simulink model "hybrid_system"  (R2026b)
settings: Solver=ode15s  StartTime=0  StopTime=200  MaxStep=0.01
undefined symbols (not defined in the file or in its folder): p
libraries: slpidlib x3
settings Model: Creator=ian  LastModifiedBy=hk

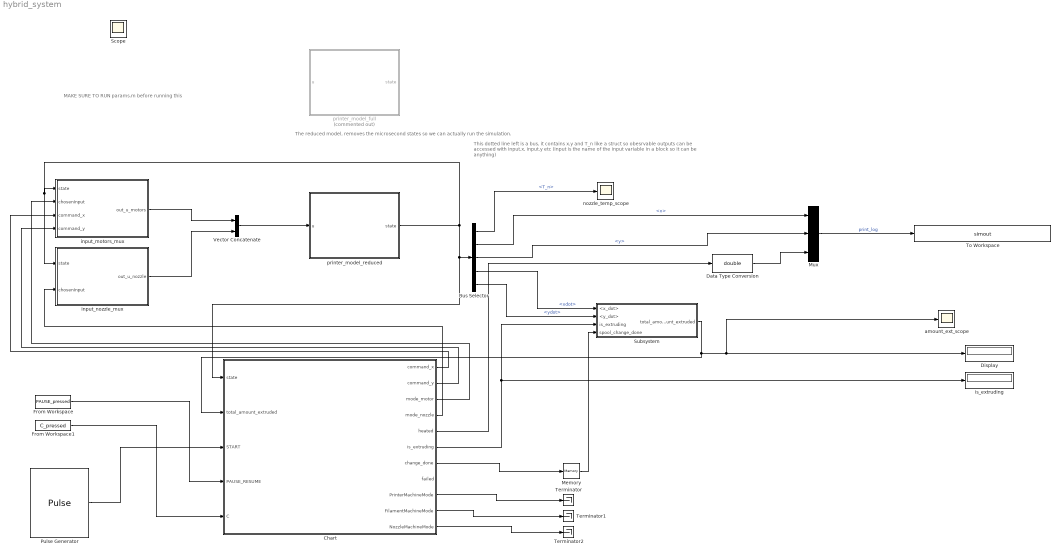
== system hybrid_system ==
  note: MAKE SURE TO RUN params.m before running this
  note: This dotted line left is a bus, it contains x,y and T_n like a struct so obesrvable outputs can be accessed with input.x, input.y etc (input is the name of the input variable in a block so it can be anything)
  note: The reduced model, removes the microsecond states so we can actually run the simulation.
  Bus Selector : BusSelector  OutputSignals=T_n,x,y,xdot,ydot
  Chart : Stateflow chart  TreatAsAtomicUnit=on
  Data Type Conversion : DataTypeConversion  OutDataTypeStr=double  SaturateOnIntegerOverflow=off  RndMeth=Floor
  Display : Display
  From Workspace : FromWorkspace  VariableName=PAUSE_pressed  Interpolate=off  OutputAfterFinalValue=Holding final value
  From Workspace1 : FromWorkspace  VariableName=C_pressed  Interpolate=off  OutputAfterFinalValue=Holding final value
  Memory : Memory
  Mux : Mux  Inputs=3
  Pulse Generator : DiscretePulseGenerator  PulseType=Time based  Period=1000  PulseWidth=0.5  PhaseDelay=1
  Subsystem : Subsystem
  Terminator : Terminator
  Terminator1 : Terminator
  Terminator2 : Terminator
  To Workspace : ToWorkspace  VariableName=simout  SaveFormat=Timeseries  SampleTime=-1
  Vector Concatenate : Concatenate
  amount_ext_scope : Scope
      settings: ActiveDisplayYMinimum=-54.541035477744657  ActiveDisplayYMaximum=83.193841611609969
  input_motors_mux : Subsystem
  input_nozzle_mux : Subsystem
  is_extruding : Display
  nozzle_temp_scope : Scope
      settings: ActiveDisplayYMinimum=258.016424423675  ActiveDisplayYMaximum=353.14399996630135
  printer_model_full : Subsystem  Commented=on
  printer_model_reduced : Subsystem
  Scope : Scope
      settings: DataLoggingVariableName=ScopeData2
  wires:
  Chart/4(mode_nozzle) -> input_nozzle_mux/2(chosenInput)
  printer_model_reduced/1(state) -> input_nozzle_mux/1(state), input_motors_mux/1(state), Chart/1(state), Bus Selector/1
  Bus Selector/1 -> nozzle_temp_scope/1  "<T_n>"
  Chart/3(mode_motor) -> input_motors_mux/2(chosenInput)
  input_nozzle_mux/1(out_u_nozzle) -> Vector Concatenate/2
  Vector Concatenate/1 -> printer_model_reduced/1(u)
  input_motors_mux/1(out_u_motors) -> Vector Concatenate/1
  Bus Selector/2 -> Mux/1  "<x>"
  Bus Selector/3 -> Mux/2  "<y>"
  Chart/5(heated) -> Data Type Conversion/1
  Data Type Conversion/1 -> Mux/3
  Mux/1 -> To Workspace/1  "print_log"
  Subsystem/1(total_amount_extruded) -> amount_ext_scope/1, Display/1, Chart/2(total_amount_extruded)
  Chart/1(command_x) -> input_motors_mux/3(command_x)
  Chart/2(command_y) -> input_motors_mux/4(command_y)
  Pulse Generator/1 -> Chart/3(START)
  From Workspace/1 -> Chart/4(PAUSE_RESUME)
  From Workspace1/1 -> Chart/5(C)
  Bus Selector/4 -> Subsystem/1(<x_dot>)  "<xdot>"
  Bus Selector/5 -> Subsystem/2(<y_dot>)  "<ydot>"
  Chart/7(change_done) -> Memory/1
  Memory/1 -> Subsystem/4(spool_change_done)
  Chart/6(is_extruding) -> is_extruding/1, Subsystem/3(is_extruding)
  Chart/9(" PrinterMachineMode") -> Terminator/1
  Chart/10(" FilamentMachineMode") -> Terminator1/1
  Chart/11(" NozzleMachineMode") -> Terminator2/1

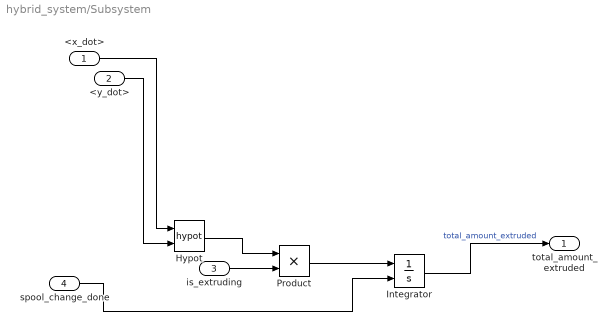
== system hybrid_system/Subsystem ==
  <x_dot> : Inport
  <y_dot> : Inport  Port=2
  is_extruding : Inport  Port=3
  spool_change_done : Inport  Port=4
  Hypot : Math  Operator=hypot
  Integrator : Integrator  ExternalReset=rising
  Product : Product
  total_amount_extruded : Outport
  wires:
  Hypot/1 -> Product/1
  Product/1 -> Integrator/1
  <y_dot>/1 -> Hypot/2
  is_extruding/1 -> Product/2
  <x_dot>/1 -> Hypot/1
  Integrator/1 -> total_amount_extruded/1  "total_amount_extruded"
  spool_change_done/1 -> Integrator/2

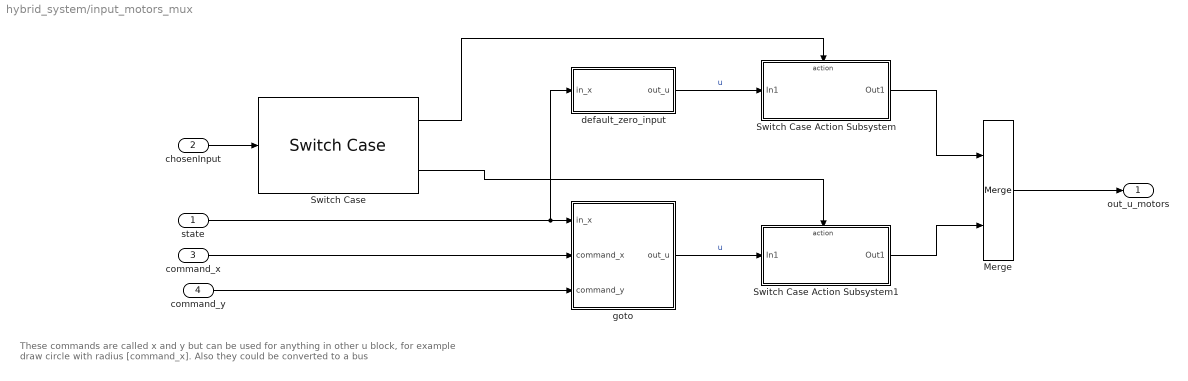
== system hybrid_system/input_motors_mux ==
  note: These commands are called x and y but can be used for anything in other u block, for example draw circle with radius [command_x]. Also they could be converted to a bus
  state : Inport
  chosenInput : Inport  Port=2  OutDataTypeStr=Enum: ModeMotors
  command_x : Inport  Port=3
  command_y : Inport  Port=4
  Merge : Merge
  Switch Case : SwitchCase  CaseConditions={ModeMotors.Off, ModeMotors.GoTo}  ShowDefaultCase=off
  Switch Case Action Subsystem : Subsystem  TreatAsAtomicUnit=on
  Switch Case Action Subsystem1 : Subsystem  TreatAsAtomicUnit=on
  default_zero_input : Subsystem
  goto : Subsystem
  out_u_motors : Outport  OutDataTypeStr=double  PortDimensions=[2 1]
  wires:
  Switch Case/2 -> Switch Case Action Subsystem1/Action
  Switch Case Action Subsystem/1(Out1) -> Merge/1
  Switch Case/1 -> Switch Case Action Subsystem/Action
  Switch Case Action Subsystem1/1(Out1) -> Merge/2
  default_zero_input/1(out_u) -> Switch Case Action Subsystem/1(In1)  "u"
  goto/1(out_u) -> Switch Case Action Subsystem1/1(In1)  "u"
  chosenInput/1 -> Switch Case/1
  Merge/1 -> out_u_motors/1
  state/1 -> default_zero_input/1(in_x), goto/1(in_x)
  command_x/1 -> goto/2(command_x)
  command_y/1 -> goto/3(command_y)

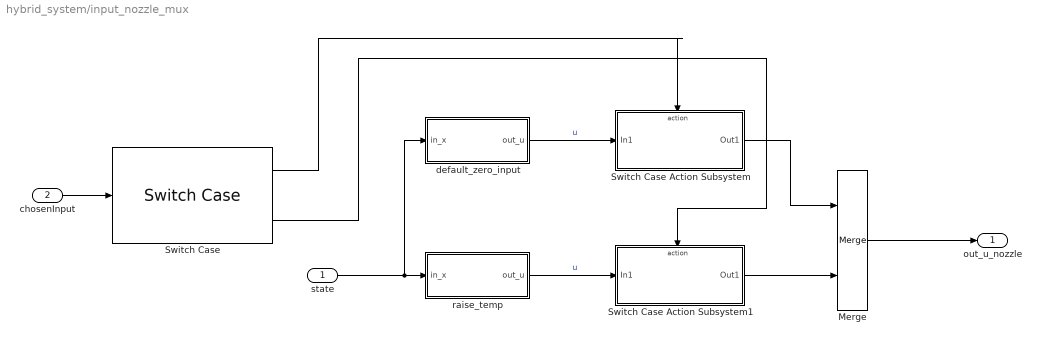
== system hybrid_system/input_nozzle_mux ==
  state : Inport
  chosenInput : Inport  Port=2  OutDataTypeStr=Enum: ModeNozzle
  Merge : Merge
  Switch Case : SwitchCase  CaseConditions={ModeNozzle.Off,ModeNozzle.HeatNozzle}  ShowDefaultCase=off
  Switch Case Action Subsystem : Subsystem  TreatAsAtomicUnit=on
  Switch Case Action Subsystem1 : Subsystem  TreatAsAtomicUnit=on
  default_zero_input : Subsystem
  raise_temp : Subsystem
  out_u_nozzle : Outport  OutDataTypeStr=double  PortDimensions=1
  wires:
  Switch Case/2 -> Switch Case Action Subsystem1/Action
  Switch Case Action Subsystem/1(Out1) -> Merge/1
  Switch Case/1 -> Switch Case Action Subsystem/Action
  Switch Case Action Subsystem1/1(Out1) -> Merge/2
  default_zero_input/1(out_u) -> Switch Case Action Subsystem/1(In1)  "u"
  raise_temp/1(out_u) -> Switch Case Action Subsystem1/1(In1)  "u"
  chosenInput/1 -> Switch Case/1
  Merge/1 -> out_u_nozzle/1
  state/1 -> default_zero_input/1(in_x), raise_temp/1(in_x)

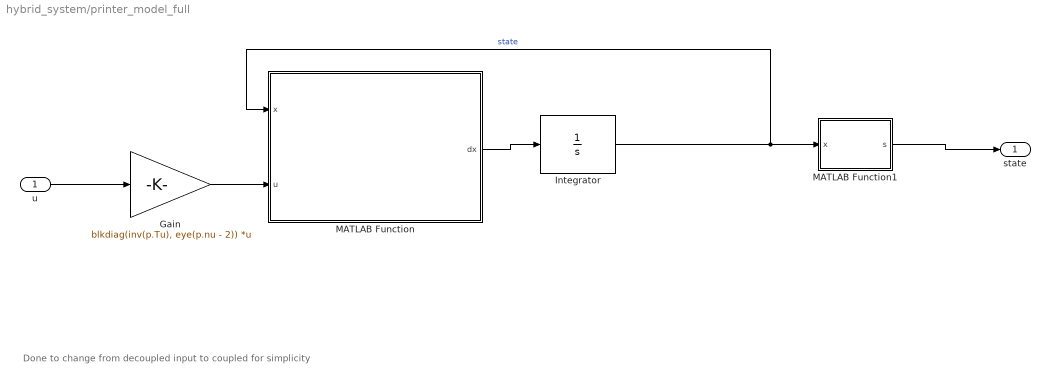
== system hybrid_system/printer_model_full ==
  note: Done to change from decoupled input to coupled for simplicity
  u : Inport  OutDataTypeStr=double  PortDimensions=[3 1]
  Gain : Gain  Gain=blkdiag(inv(p.Tu), eye(p.nu - 2))  Multiplication=Matrix(K*u)
  Integrator : Integrator  InitialCondition=p.x0
  MATLAB Function : MATLAB Function  TreatAsAtomicUnit=on
  MATLAB Function1 : MATLAB Function  TreatAsAtomicUnit=on
  state : Outport  OutDataTypeStr=Bus: PlantState
  wires:
  MATLAB Function/1(dx) -> Integrator/1
  Integrator/1 -> MATLAB Function1/1(x), MATLAB Function/1(x)  "state"
  MATLAB Function1/1(s) -> state/1
  Gain/1 -> MATLAB Function/2(u)
  u/1 -> Gain/1

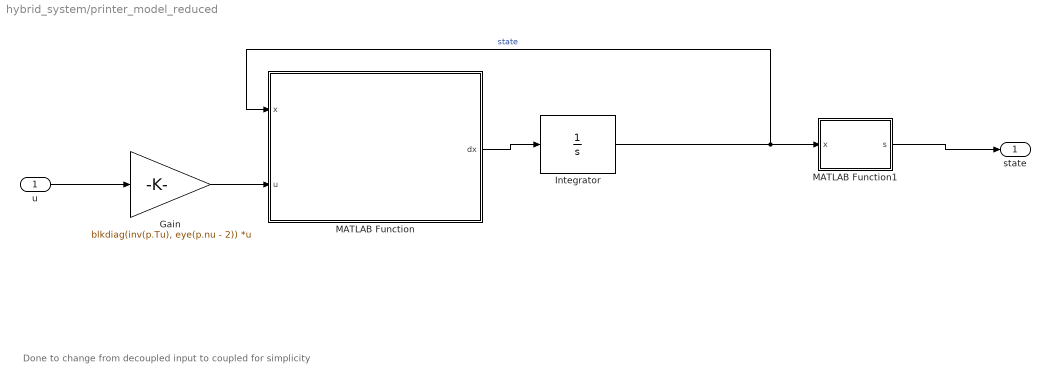
== system hybrid_system/printer_model_reduced ==
  note: Done to change from decoupled input to coupled for simplicity
  u : Inport
  Gain : Gain  Gain=blkdiag(inv(p.Tu), eye(p.nu - 2))  Multiplication=Matrix(K*u)
  Integrator : Integrator  InitialCondition=p.red.x0
  MATLAB Function : MATLAB Function  TreatAsAtomicUnit=on
  MATLAB Function1 : MATLAB Function  TreatAsAtomicUnit=on
  state : Outport  OutDataTypeStr=Bus: PlantState
  wires:
  MATLAB Function/1(dx) -> Integrator/1
  Integrator/1 -> MATLAB Function1/1(x), MATLAB Function/1(x)  "state"
  MATLAB Function1/1(s) -> state/1
  Gain/1 -> MATLAB Function/2(u)
  u/1 -> Gain/1

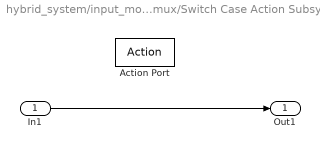
== system hybrid_system/input_motors_mux/Switch Case Action Subsystem ==
  In1 : Inport
  Action Port : ActionPort  ActionPortLabel=case [ Off ]:
  Out1 : Outport
  wires:
  In1/1 -> Out1/1

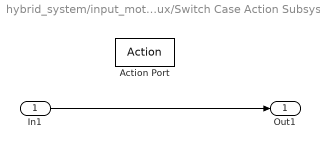
== system hybrid_system/input_motors_mux/Switch Case Action Subsystem1 ==
  In1 : Inport
  Action Port : ActionPort  ActionPortLabel=case [ GoTo ]:
  Out1 : Outport
  wires:
  In1/1 -> Out1/1

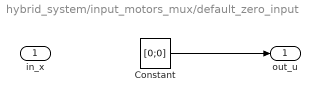
== system hybrid_system/input_motors_mux/default_zero_input ==
  in_x : Inport
  Constant : Constant  Value=[0;0]
  out_u : Outport
  wires:
  Constant/1 -> out_u/1

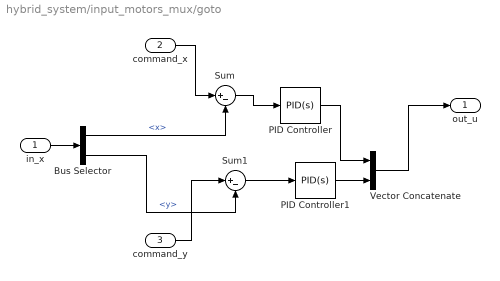
== system hybrid_system/input_motors_mux/goto ==
  in_x : Inport
  command_x : Inport  Port=2
  command_y : Inport  Port=3
  Bus Selector : BusSelector  OutputSignals=x,y
  PID Controller : slpidlib/PID Controller  Controller=PID  Form=Parallel  TimeDomain=Continuous-time  UseExternalTs=off  SampleTime=-1  IntegratorMethod=Forward Euler  FilterMethod=Forward Euler  ControllerParametersSource=internal  P=10  I=0  UseKiTs=off  D=0  UseExternalDerivativeSource=off  N=100  UseFilter=on  TunerSelectOption=Transfer Function Based (PID Tuner App)  InitialConditionSource=internal  InitialConditionForIntegrator=0  InitialConditionForFilter=0  DifferentiatorICPrevScaledInput=0  ExternalReset=none  TrackingMode=off  Kt=1  LimitOutput=on  SatLimitsSource=internal  UpperSaturationLimit=15  LowerSaturationLimit=-15  LinearizeAsGain=on  AntiWindupMode=none  Kb=1  LimitIntegrator=off  UpperIntegratorSaturationLimit=inf  LowerIntegratorSaturationLimit=-inf  POutMin=[]  POutMax=[]  IOutMin=[]  IOutMax=[]  DOutMin=[]  DOutMax=[]  NOutMin=[]  NOutMax=[]  SumOutMin=[]  SumOutMax=[]  SaturationOutMin=[]  SaturationOutMax=[]  PParamMin=[]  PParamMax=[]  IParamMin=[]  IParamMax=[]  DParamMin=[]  DParamMax=[]  NParamMin=[]  NParamMax=[]  KbParamMin=[]  KbParamMax=[]  KtParamMin=[]  KtParamMax=[]  KbOutMin=[]  KbOutMax=[]  KtOutMin=[]  KtOutMax=[]  IntegratorOutMin=[]  IntegratorOutMax=[]  FilterOutMin=[]  FilterOutMax=[]  SumI1OutMin=[]  SumI1OutMax=[]  SumI2OutMin=[]  SumI2OutMax=[]  SumI3OutMin=[]  SumI3OutMax=[]  SumI4OutMin=[]  SumI4OutMax=[]  SumDOutMin=[]  SumDOutMax=[]  DifferentiatorOutMin=[]  DifferentiatorOutMax=[]  FilterDiffOutCoefMin=[]  FilterDiffOutCoefMax=[]  ReciprocalOutMin=[]  ReciprocalOutMax=[]  SumDenOutMin=[]  SumDenOutMax=[]  SumNumOutMin=[]  SumNumOutMax=[]  DivideOutMin=[]  DivideOutMax=[]  UdiffTsProdOutMin=[]  UdiffTsProdOutMax=[]  NTsProdOutMin=[]  NTsProdOutMax=[]  UintegralTsProdOutMin=[]  UintegralTsProdOutMax=[]  UngainTsProdOutMin=[]  UngainTsProdOutMax=[]  ClampingZeroOutDataTypeStr=Inherit: Inherit via back propagation  ClampingZeroOutMin=[]  ClampingZeroOutMax=[]  FilterDenConstantOutDataTypeStr=Inherit: Inherit via back propagation  FilterDenConstantOutMin=[]  FilterDenConstantOutMax=[]  PCopyOutDataTypeStr=Inherit: Inherit via back propagation  PCopyOutMin=[]  PCopyOutMax=[]  NCopyOutDataTypeStr=Inherit: Inherit via back propagation  NCopyOutMin=[]  NCopyOutMax=[]  IntegratorContinuousStateAttributes=''  IntegratorStateMustResolveToSignalObject=off  IntegratorRTWStateStorageClass=Auto  FilterContinuousStateAttributes=''  FilterStateMustResolveToSignalObject=off  FilterRTWStateStorageClass=Auto  ParallelPVariant=InternalParameters  IdealPVariant=Disabled  IVariant=InternalParameters  DVariant=InternalParameters  IntegratorVariant=Continuous  SatVariant=Enabled  AWVariant=Passthrough  PCopyVariant=Disabled  TRVariant=Disabled  FdbkBlocksVariant=Forward  IdealPFdbkVariant=Disabled  SatFdbkVariant=Disabled  DerivativeFilterVariant=ContFilter  NVariant=InternalParameters  NCopyVariant=Disabled  FilterICVariant=InternalICsFilter  IntegratorICVariant=InternalICs  ExternalResetVariant=Disabled  TRSumVariant=Passthrough  SumFdbkVariant=Disabled  SumVariant=Sum_PID  TsampFilterVariant=InternalTs  TsampNgainVariant=Passthrough  TsampIntegralVariant=Disabled_SignalSpec  ExternalSaturationOutDataTypeStr=Inherit: Same as second input  DerivativeSourceVariant=ErrorSignal  PreIntVariant=InternalPreInt
  PID Controller1 : slpidlib/PID Controller  Controller=PID  Form=Parallel  TimeDomain=Continuous-time  UseExternalTs=off  SampleTime=-1  IntegratorMethod=Forward Euler  FilterMethod=Forward Euler  ControllerParametersSource=internal  P=10  I=0  UseKiTs=off  D=0  UseExternalDerivativeSource=off  N=100  UseFilter=on  TunerSelectOption=Transfer Function Based (PID Tuner App)  InitialConditionSource=internal  InitialConditionForIntegrator=0  InitialConditionForFilter=0  DifferentiatorICPrevScaledInput=0  ExternalReset=none  TrackingMode=off  Kt=1  LimitOutput=on  SatLimitsSource=internal  UpperSaturationLimit=15  LowerSaturationLimit=-15  LinearizeAsGain=on  AntiWindupMode=none  Kb=1  LimitIntegrator=off  UpperIntegratorSaturationLimit=inf  LowerIntegratorSaturationLimit=-inf  POutMin=[]  POutMax=[]  IOutMin=[]  IOutMax=[]  DOutMin=[]  DOutMax=[]  NOutMin=[]  NOutMax=[]  SumOutMin=[]  SumOutMax=[]  SaturationOutMin=[]  SaturationOutMax=[]  PParamMin=[]  PParamMax=[]  IParamMin=[]  IParamMax=[]  DParamMin=[]  DParamMax=[]  NParamMin=[]  NParamMax=[]  KbParamMin=[]  KbParamMax=[]  KtParamMin=[]  KtParamMax=[]  KbOutMin=[]  KbOutMax=[]  KtOutMin=[]  KtOutMax=[]  IntegratorOutMin=[]  IntegratorOutMax=[]  FilterOutMin=[]  FilterOutMax=[]  SumI1OutMin=[]  SumI1OutMax=[]  SumI2OutMin=[]  SumI2OutMax=[]  SumI3OutMin=[]  SumI3OutMax=[]  SumI4OutMin=[]  SumI4OutMax=[]  SumDOutMin=[]  SumDOutMax=[]  DifferentiatorOutMin=[]  DifferentiatorOutMax=[]  FilterDiffOutCoefMin=[]  FilterDiffOutCoefMax=[]  ReciprocalOutMin=[]  ReciprocalOutMax=[]  SumDenOutMin=[]  SumDenOutMax=[]  SumNumOutMin=[]  SumNumOutMax=[]  DivideOutMin=[]  DivideOutMax=[]  UdiffTsProdOutMin=[]  UdiffTsProdOutMax=[]  NTsProdOutMin=[]  NTsProdOutMax=[]  UintegralTsProdOutMin=[]  UintegralTsProdOutMax=[]  UngainTsProdOutMin=[]  UngainTsProdOutMax=[]  ClampingZeroOutDataTypeStr=Inherit: Inherit via back propagation  ClampingZeroOutMin=[]  ClampingZeroOutMax=[]  FilterDenConstantOutDataTypeStr=Inherit: Inherit via back propagation  FilterDenConstantOutMin=[]  FilterDenConstantOutMax=[]  PCopyOutDataTypeStr=Inherit: Inherit via back propagation  PCopyOutMin=[]  PCopyOutMax=[]  NCopyOutDataTypeStr=Inherit: Inherit via back propagation  NCopyOutMin=[]  NCopyOutMax=[]  IntegratorContinuousStateAttributes=''  IntegratorStateMustResolveToSignalObject=off  IntegratorRTWStateStorageClass=Auto  FilterContinuousStateAttributes=''  FilterStateMustResolveToSignalObject=off  FilterRTWStateStorageClass=Auto  ParallelPVariant=InternalParameters  IdealPVariant=Disabled  IVariant=InternalParameters  DVariant=InternalParameters  IntegratorVariant=Continuous  SatVariant=Enabled  AWVariant=Passthrough  PCopyVariant=Disabled  TRVariant=Disabled  FdbkBlocksVariant=Forward  IdealPFdbkVariant=Disabled  SatFdbkVariant=Disabled  DerivativeFilterVariant=ContFilter  NVariant=InternalParameters  NCopyVariant=Disabled  FilterICVariant=InternalICsFilter  IntegratorICVariant=InternalICs  ExternalResetVariant=Disabled  TRSumVariant=Passthrough  SumFdbkVariant=Disabled  SumVariant=Sum_PID  TsampFilterVariant=InternalTs  TsampNgainVariant=Passthrough  TsampIntegralVariant=Disabled_SignalSpec  ExternalSaturationOutDataTypeStr=Inherit: Same as second input  DerivativeSourceVariant=ErrorSignal  PreIntVariant=InternalPreInt
  Sum : Sum  Inputs=|+-
  Sum1 : Sum  Inputs=|+-
  Vector Concatenate : Concatenate
  out_u : Outport
  wires:
  in_x/1 -> Bus Selector/1
  Bus Selector/1 -> Sum/2  "<x>"
  command_x/1 -> Sum/1
  Sum/1 -> PID Controller/1
  PID Controller/1 -> Vector Concatenate/1
  command_y/1 -> Sum1/1
  Bus Selector/2 -> Sum1/2  "<y>"
  Sum1/1 -> PID Controller1/1
  PID Controller1/1 -> Vector Concatenate/2
  Vector Concatenate/1 -> out_u/1

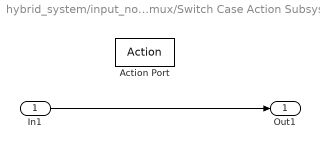
== system hybrid_system/input_nozzle_mux/Switch Case Action Subsystem ==
  In1 : Inport
  Action Port : ActionPort  ActionPortLabel=case [ Off ]:
  Out1 : Outport
  wires:
  In1/1 -> Out1/1

== system hybrid_system/input_nozzle_mux/Switch Case Action Subsystem1 ==
  In1 : Inport
  Action Port : ActionPort  ActionPortLabel=case [ HeatNozzle ]:
  Out1 : Outport
  wires:
  In1/1 -> Out1/1

== system hybrid_system/input_nozzle_mux/default_zero_input ==
  in_x : Inport
  Constant : Constant  Value=[0]
  out_u : Outport
  wires:
  Constant/1 -> out_u/1

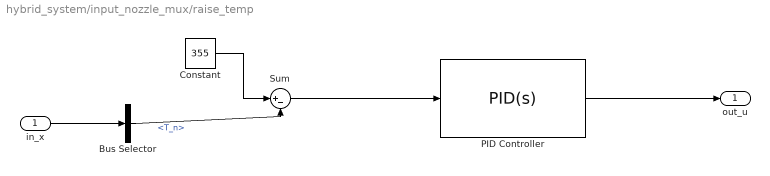
== system hybrid_system/input_nozzle_mux/raise_temp ==
  in_x : Inport
  Bus Selector : BusSelector  OutputSignals=T_n
  Constant : Constant  Value=355
  PID Controller : slpidlib/PID Controller  Controller=PID  Form=Parallel  TimeDomain=Continuous-time  UseExternalTs=off  SampleTime=1  IntegratorMethod=Forward Euler  FilterMethod=Forward Euler  ControllerParametersSource=internal  P=10  I=0  UseKiTs=on  D=20  UseExternalDerivativeSource=off  N=100  UseFilter=on  TunerSelectOption=Transfer Function Based (PID Tuner App)  InitialConditionSource=internal  InitialConditionForIntegrator=0  InitialConditionForFilter=0  DifferentiatorICPrevScaledInput=0  ExternalReset=none  TrackingMode=off  Kt=1  LimitOutput=on  SatLimitsSource=internal  UpperSaturationLimit=25  LowerSaturationLimit=0  LinearizeAsGain=on  AntiWindupMode=none  Kb=1  LimitIntegrator=off  UpperIntegratorSaturationLimit=inf  LowerIntegratorSaturationLimit=-inf  POutMin=[]  POutMax=[]  IOutMin=[]  IOutMax=[]  DOutMin=[]  DOutMax=[]  NOutMin=[]  NOutMax=[]  SumOutMin=[]  SumOutMax=[]  SaturationOutMin=[]  SaturationOutMax=[]  PParamMin=[]  PParamMax=[]  IParamMin=[]  IParamMax=[]  DParamMin=[]  DParamMax=[]  NParamMin=[]  NParamMax=[]  KbParamMin=[]  KbParamMax=[]  KtParamMin=[]  KtParamMax=[]  KbOutMin=[]  KbOutMax=[]  KtOutMin=[]  KtOutMax=[]  IntegratorOutMin=[]  IntegratorOutMax=[]  FilterOutMin=[]  FilterOutMax=[]  SumI1OutMin=[]  SumI1OutMax=[]  SumI2OutMin=[]  SumI2OutMax=[]  SumI3OutMin=[]  SumI3OutMax=[]  SumI4OutMin=[]  SumI4OutMax=[]  SumDOutMin=[]  SumDOutMax=[]  DifferentiatorOutMin=[]  DifferentiatorOutMax=[]  FilterDiffOutCoefMin=[]  FilterDiffOutCoefMax=[]  ReciprocalOutMin=[]  ReciprocalOutMax=[]  SumDenOutMin=[]  SumDenOutMax=[]  SumNumOutMin=[]  SumNumOutMax=[]  DivideOutMin=[]  DivideOutMax=[]  UdiffTsProdOutMin=[]  UdiffTsProdOutMax=[]  NTsProdOutMin=[]  NTsProdOutMax=[]  UintegralTsProdOutMin=[]  UintegralTsProdOutMax=[]  UngainTsProdOutMin=[]  UngainTsProdOutMax=[]  ClampingZeroOutDataTypeStr=Inherit: Inherit via back propagation  ClampingZeroOutMin=[]  ClampingZeroOutMax=[]  FilterDenConstantOutDataTypeStr=Inherit: Inherit via back propagation  FilterDenConstantOutMin=[]  FilterDenConstantOutMax=[]  PCopyOutDataTypeStr=Inherit: Inherit via back propagation  PCopyOutMin=[]  PCopyOutMax=[]  NCopyOutDataTypeStr=Inherit: Inherit via back propagation  NCopyOutMin=[]  NCopyOutMax=[]  IntegratorContinuousStateAttributes=''  IntegratorStateMustResolveToSignalObject=off  IntegratorRTWStateStorageClass=Auto  FilterContinuousStateAttributes=''  FilterStateMustResolveToSignalObject=off  FilterRTWStateStorageClass=Auto  ParallelPVariant=InternalParameters  IdealPVariant=Disabled  IVariant=InternalParameters  DVariant=InternalParameters  IntegratorVariant=Continuous  SatVariant=Enabled  AWVariant=Passthrough  PCopyVariant=Disabled  TRVariant=Disabled  FdbkBlocksVariant=Forward  IdealPFdbkVariant=Disabled  SatFdbkVariant=Disabled  DerivativeFilterVariant=ContFilter  NVariant=InternalParameters  NCopyVariant=Disabled  FilterICVariant=InternalICsFilter  IntegratorICVariant=InternalICs  ExternalResetVariant=Disabled  TRSumVariant=Passthrough  SumFdbkVariant=Disabled  SumVariant=Sum_PID  TsampFilterVariant=InternalTs  TsampNgainVariant=Passthrough  TsampIntegralVariant=Disabled_SignalSpec  ExternalSaturationOutDataTypeStr=Inherit: Same as second input  DerivativeSourceVariant=ErrorSignal  PreIntVariant=InternalPreInt
  Sum : Sum  Inputs=|+-
  out_u : Outport
  wires:
  PID Controller/1 -> out_u/1
  in_x/1 -> Bus Selector/1
  Bus Selector/1 -> Sum/2  "<T_n>"
  Constant/1 -> Sum/1
  Sum/1 -> PID Controller/1

== matlab function hybrid_system/printer_model_full/MATLAB Function1 ==
  data: x input; s output Bus: PlantState; p parameter
function s = to_bus(x, p)
%TO_BUS  Convert the state vector to a PlantState bus (struct with named fields).
s.x    = x(p.idx.x);
s.y    = x(p.idx.y);
s.T_n  = x(p.idx.T_n);
end

== matlab function hybrid_system/printer_model_full/MATLAB Function ==
  data: x input; u input; dx output; p parameter
function dx = f(x, u, p)
dx = sys(x, u, p);
end

== stateflow chart hybrid_system/Chart ==
  state NozzleMachine [parallel]
    settings: executionOrder=1
    state Cooling
      entry: mode_nozzle = ModeNozzle.Off
    state HeatingUp
      entry: mode_nozzle = ModeNozzle.HeatNozzle
    state cooled_but_not_supposed_to
      %ERROR
    state Heated
      entry: heated=true
    state Cool
      entry: heated=false
    state too_hot
      %ERROR
    Cool -> HeatingUp : [request_heated_nozzle]
    Cooling -> Cool : [duration(state.T_n < 350) > 1]
    Heated -> Cooling [order 3] : [~request_heated_nozzle]
    HeatingUp -> Heated : [duration(state.T_n >=350) > 1]
    Heated -> cooled_but_not_supposed_to [order 1] : [state.T_n < 350]
    (default) -> Cool
    Heated -> too_hot [order 2] : [state.T_n > 370]
  state PrinterMachine [parallel]
    during: arrived = abs(state.x - command_x) < p.tol && abs(state.y - command_y) < p.tol;
    F = total_amount_extruded >=p.fil_max;
    at_wall = abs(state.x) >= p.L_bed - 1e-4 && abs(state.xdot) < 0.0005;
    settings: executionOrder=2
    state COMPLETED
      entry:
      mode_motor = ModeMotors.Off;
      is_extruding = false;
      request_heated_nozzle = false;
      fprintf('%.1f s:Print Complete \n', getSimulationTime());
      fprintf('%.1f s: Amt extruded on completion = %.3f m\n', getSimulationTime(), total_amount_extruded);
    state IN_PROGRESS
      entry:
      request_heated_nozzle = true;
      fprintf('%.1f s: Printing In Progress \n', getSimulationTime());
      state PRINT_PATH
        entry:
        mode_motor = ModeMotors.GoTo;
        is_extruding = true;
        command_x = p.path(k, 1);
        command_y = p.path(k, 2);
        fprintf('%.1f s: Print In Prog \n', getSimulationTime());
      state TRAVEL_TO_START
        entry:
        mode_motor = ModeMotors.GoTo;
        is_extruding = false;
        command_x =p.path(max(k-1,1),1);
        command_y = p.path(max(k-1,1),2);
        fprintf('%.1f s: Going to Home Position \n', getSimulationTime());
      state WAIT_HOT
        entry:
        mode_motor = ModeMotors.Off;
        is_extruding = false;
      PRINT_PATH -> PRINT_PATH [order 1] : [k < p.n_path && arrived]{k = k + 1;}
      TRAVEL_TO_START -> PRINT_PATH [order 1] : [duration(arrived) > 0.5 && ~failed]{k=max(k,2)}
      PRINT_PATH -> TRAVEL_TO_START [order 4] : [at_wall]{fprintf('%.1f s: At wall, going home \n', getSimulationTime());
          | failed=true;}
      (default) -> WAIT_HOT
      WAIT_HOT -> TRAVEL_TO_START : [heated]
    state IDLE
      entry: mode_motor=ModeMotors.Off;
      is_extruding = false;
      command_x = 0;
      command_y=0;
      request_heated_nozzle = false;
      paused = false;
    state FAILED
      entry:mode_motor = ModeMotors.Off;
      is_extruding = false;
      request_heated_nozzle = false;
      fprintf('%.1f s: Print Failed \n', getSimulationTime());
    state PAUSED
      entry:
      paused = true;
      saved_x = state.x;
      saved_y = state.y;
      mode_motor = ModeMotors.GoTo;
      command_x = saved_x;
      command_y = saved_y;
      is_extruding = false;
      request_heated_nozzle=false;
      fprintf('%.1f s: Paused \n', getSimulationTime());
    (default) -> PrinterMachine.IDLE
    PRINT_PATH -> FAILED [order 3] : [at_wall]{fprintf('%.1f s: At wall, going home \n', getSimulationTime());}
    PRINT_PATH -> COMPLETED [order 2] : [k == p.n_path && duration(arrived) > 0.5]
    PrinterMachine.IDLE -> IN_PROGRESS : [START==1]{fprintf('%.1f s: Print Initiated \n', getSimulationTime());
        | }
    TRAVEL_TO_START -> FAILED [order 2] : [duration(arrived) > 0.5 && ~failed]
    IN_PROGRESS -> PAUSED : [hasChangedTo(PAUSE_RESUME, 1) || hasChangedTo(C, 1) || F]
    PAUSED -> IN_PROGRESS : [(hasChangedTo(PAUSE_RESUME, 1)  || change_done) && ~change_active]{paused=false;}
  state FilamentMachine [parallel]
    settings: executionOrder=3
    state WIPING
      entry:
      is_extruding=true;
      command_x=p.wipe_x + 0.02
    state MOVING_TO_WIPE
      entry:
      mode_motor = ModeMotors.GoTo;
      command_x = p.wipe_x;
      command_y = p.wipe_y;
      is_extruding = false;
    state NOZZLE_COOLING
      entry:
      is_extruding = false;
      request_heated_nozzle = false;
    state IDLE
      entry:
      change_active=false;
    state NOZZLE_HEATING
      entry:
      is_extruding = false;
      request_heated_nozzle = true;
    state LOADING_FILAMENT
      entry:fprintf('%.1f s: loading\n', getSimulationTime());
    state READY_TO_RESUME
      entry:
      command_x = saved_x;
      command_y = saved_y;
      is_extruding = false;
    WIPING -> NOZZLE_COOLING : [after(p.t_wipe,sec)]{fprintf('%.1f s: Wiped Successful\n', getSimulationTime());}
    MOVING_TO_WIPE -> WIPING : [duration(arrived)>0.5]{fprintf('%.1f s: Moving to Wiping Location Successful\n', getSimulationTime());}
    FilamentMachine.IDLE -> MOVING_TO_WIPE : [hasChangedTo(C, 1) || F]{change_active = true;change_done=false;
        | fprintf('%.1f s: Filament Change Triggered\n', getSimulationTime());}
    NOZZLE_COOLING -> LOADING_FILAMENT : [~heated]{fprintf('%.1f s: Nozzle Cooled\n', getSimulationTime());}
    (default) -> FilamentMachine.IDLE
    NOZZLE_HEATING -> FilamentMachine.IDLE [order 2] : [heated && ~paused]{change_done=true;
        | fprintf('%.1f s: Filament Change Done\n', getSimulationTime());}
    READY_TO_RESUME -> FilamentMachine.IDLE : [duration(arrived)>0.5]{change_done=true;
        | fprintf('%.1f s: Filament Change Done\n', getSimulationTime());}
    NOZZLE_HEATING -> READY_TO_RESUME [order 1] : [heated && paused]
    LOADING_FILAMENT -> NOZZLE_HEATING : [after(p.t_load,sec)]{fprintf('%.1f s: Loaded Filament\n', getSimulationTime());}
  data: command_x output; command_y output; mode_motor output Enum: ModeMotors; state input; mode_nozzle output Enum: ModeNozzle; request_heated_nozzle local =false; heated output; start_drawing local double =1; total_amount_extruded input; is_extruding output; START input; saved_x local; saved_y local; retries_left local; p parameter; arrived local =false; k local =2; PAUSE_RESUME input; C input; change_active local; paused local; change_done output; data local; F local; at_wall local; failed output =false; PrinterMachineMode output Enum: PrinterMachineModeType; FilamentMachineMode output Enum: FilamentMachineModeType; NozzleMachineMode output Enum: NozzleMachineModeType

== matlab function hybrid_system/printer_model_reduced/MATLAB Function ==
  data: x input; u input; dx output; p parameter
function dx = f(x, u, p)
dx = sys_reduced(x, u, p);
end

== matlab function hybrid_system/printer_model_reduced/MATLAB Function1 ==
  data: x input; s output Bus: PlantState; p parameter
function s = to_bus(x, p)
%TO_BUS  Convert the state vector to a PlantState bus (struct with named fields).
s.x    = x(p.red.idx.x);
s.y    = x(p.red.idx.y);
s.xdot = x(p.red.idx.xdot);
s.ydot = x(p.red.idx.ydot);
s.T_n  = x(p.red.idx.T_n);
end
